simulink model "tb_elec_plant"  (R2026b)
values from neighbouring files (symbols this model uses):
  P = evalin('base', 'P')    [elec_harness.m]    (also in mcu_can1_roundtrip.m; mcu_can2_roundtrip.m; mcu_cl_input.m; mcu_ctrl_harness.m)
  Ts = prm(1)    [mcu_cl_track_dyn.m]    (also in mcu_ctrl_harness.m = evalin('base', tsExpr))
undefined symbols (not defined in the file or in its folder): EStop_Ch1_OK, EStop_Ch2_OK, G_solar, K1_Closed, K2_Closed, Key_On, Rail_12V_OK, Rail_24V_OK, Rail_3V3_OK, Rail_5V_OK, Safety_HV_OK, Safety_OK, T_amb, V_12V_V, V_24V_V, V_3V3_V, V_5V_V, V_bus_V, V_pack_V
settings Model: Creator=aomar  LastModifiedBy=aomar

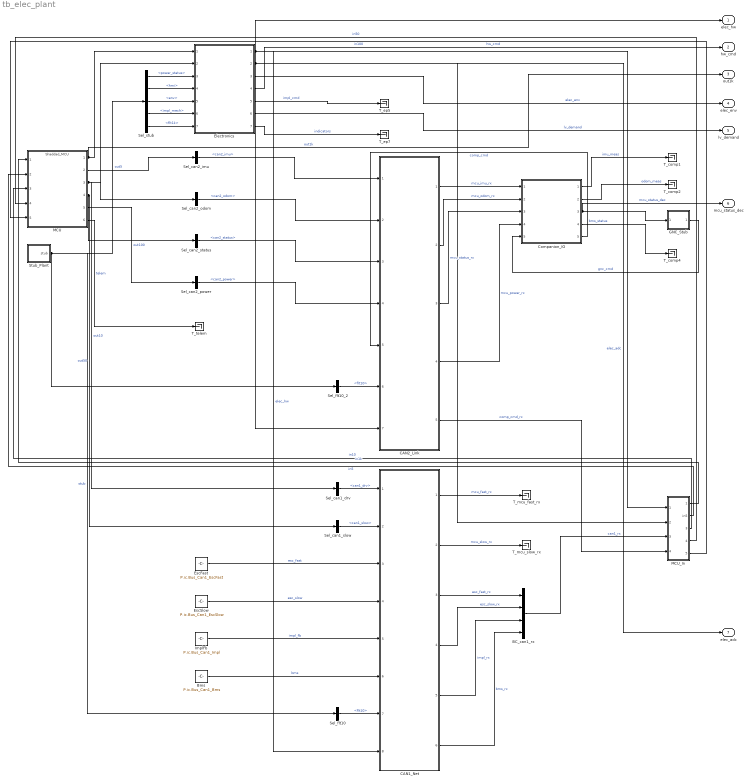
== system tb_elec_plant ==
  BC_can1_rx : BusCreator  Inputs=4
  Bms : Constant  Value=P.ic.Bus_Can1_Bms  OutDataTypeStr=Bus: Bus_Can1_Bms  SampleTime=Ts.hk
  CAN1_Net : Subsystem  ReferencedSubsystem=CAN1_Net_Sim
  CAN2_Link : Subsystem  ReferencedSubsystem=Link_MCU_GNC
  Companion_IO : Subsystem  ReferencedSubsystem=companion_io
  Electronics : Subsystem  ReferencedSubsystem=Electronics_Plant
  EscFast : Constant  Value=P.ic.Bus_Can1_EscFast  OutDataTypeStr=Bus: Bus_Can1_EscFast  SampleTime=Ts.ctrl
  EscSlow : Constant  Value=P.ic.Bus_Can1_EscSlow  OutDataTypeStr=Bus: Bus_Can1_EscSlow  SampleTime=Ts.comm
  GNC_Stub : Subsystem
  ImplFb : Constant  Value=P.ic.Bus_Can1_Impl  OutDataTypeStr=Bus: Bus_Can1_Impl  SampleTime=Ts.comm
  MCU : ModelReference  ModelNameDialog=Shaddad_MCU  SimulationMode=Normal  ModelReferenceVersion=1.1
  MCU_In : Subsystem
  Sel_can1_drv : BusSelector  OutputSignals=can1_drv
  Sel_can1_slow : BusSelector  OutputSignals=can1_slow
  Sel_can2_imu : BusSelector  OutputSignals=can2_imu
  Sel_can2_odom : BusSelector  OutputSignals=can2_odom
  Sel_can2_power : BusSelector  OutputSignals=can2_power
  Sel_can2_status : BusSelector  OutputSignals=can2_status
  Sel_flt10 : BusSelector  OutputSignals=flt10
  Sel_flt10_2 : BusSelector  OutputSignals=flt10
  Sel_stub : BusSelector  OutputSignals=power_status,hmi,env,impl_mech,flt1k
  Stub_Plant : Subsystem
  T_comp1 : Terminator
  T_comp2 : Terminator
  T_comp4 : Terminator
  T_ep5 : Terminator
  T_ep7 : Terminator
  T_mcu_fast_rx : Terminator
  T_mcu_slow_rx : Terminator
  T_telem : Terminator
  elec_hw : Outport  OutDataTypeStr=Bus: Bus_ElecHwIn
  hw_cmd : Outport  Port=2  OutDataTypeStr=Bus: Bus_PowerHwCmd
  out1k : Outport  Port=3  OutDataTypeStr=Bus: Bus_McuOut1k
  elec_env : Outport  Port=4  OutDataTypeStr=Bus: Bus_ElecEnv
  lv_demand : Outport  Port=5  OutDataTypeStr=Bus: Bus_LV_LoadDemand
  mcu_status_dec : Outport  Port=6  OutDataTypeStr=Bus: Bus_McuStatus
  elec_adc : Outport  Port=7  OutDataTypeStr=Bus: Bus_ElecAdc
  wires:
  Stub_Plant/1(stub) -> Sel_flt10/1, Sel_stub/1, Sel_flt10_2/1  "stub"
  MCU/1 -> Electronics/1, out1k/1  "out1k"
  MCU/2 -> Sel_can2_imu/1  "out5"
  MCU/5 -> Sel_can2_power/1  "out100"
  MCU/6 -> T_telem/1  "telem"
  Sel_stub/1 -> Electronics/3  "<power_status>"
  Sel_stub/2 -> Electronics/4  "<hmi>"
  Sel_stub/3 -> Electronics/5  "<env>"
  Sel_stub/4 -> Electronics/6  "<impl_mech>"
  Sel_stub/5 -> Electronics/7  "<flt1k>"
  Sel_can2_imu/1 -> CAN2_Link/1  "<can2_imu>"
  Sel_can2_odom/1 -> CAN2_Link/2  "<can2_odom>"
  Sel_can2_status/1 -> CAN2_Link/3  "<can2_status>"
  Sel_can2_power/1 -> CAN2_Link/4  "<can2_power>"
  EscFast/1 -> CAN1_Net/3  "esc_fast"
  EscSlow/1 -> CAN1_Net/4  "esc_slow"
  ImplFb/1 -> CAN1_Net/5  "impl_fb"
  Bms/1 -> CAN1_Net/6  "bms"
  Electronics/1 -> CAN1_Net/8, MCU_In/1(elec_hw), CAN2_Link/7, elec_hw/1  "elec_hw"
  Electronics/2 -> elec_adc/1, MCU_In/2(elec_adc)  "elec_adc"
  Electronics/3 -> elec_env/1  "elec_env"
  Electronics/4 -> hw_cmd/1  "hw_cmd"
  Electronics/5 -> T_ep5/1  "impl_cmd"
  Electronics/6 -> lv_demand/1  "lv_demand"
  Electronics/7 -> T_ep7/1  "indicators"
  Sel_flt10_2/1 -> CAN2_Link/6  "<flt10>"
  Sel_can1_drv/1 -> CAN1_Net/1  "<can1_drv>"
  Sel_can1_slow/1 -> CAN1_Net/2  "<can1_slow>"
  Sel_flt10/1 -> CAN1_Net/7  "<flt10>"
  CAN2_Link/1 -> Companion_IO/1  "mcu_imu_rx"
  CAN2_Link/2 -> Companion_IO/2  "mcu_odom_rx"
  CAN2_Link/3 -> Companion_IO/3  "mcu_status_rx"
  CAN2_Link/4 -> Companion_IO/4  "mcu_power_rx"
  CAN2_Link/5 -> MCU_In/4(comp)  "comp_cmd_rx"
  CAN1_Net/1 -> T_mcu_fast_rx/1  "mcu_fast_rx"
  CAN1_Net/2 -> T_mcu_slow_rx/1  "mcu_slow_rx"
  CAN1_Net/3 -> BC_can1_rx/1  "esc_fast_rx"
  CAN1_Net/4 -> BC_can1_rx/2  "esc_slow_rx"
  CAN1_Net/5 -> BC_can1_rx/3  "impl_rx"
  CAN1_Net/6 -> BC_can1_rx/4  "bms_rx"
  BC_can1_rx/1 -> MCU_In/3(can1)  "can1_rx"
  Companion_IO/1 -> T_comp1/1  "imu_meas"
  Companion_IO/2 -> T_comp2/1  "odom_meas"
  Companion_IO/3 -> GNC_Stub/1(mcu_status), mcu_status_dec/1  "mcu_status_dec"
  Companion_IO/4 -> T_comp4/1  "bms_status"
  Companion_IO/5 -> CAN2_Link/5  "comp_cmd"
  GNC_Stub/1(gnc_cmd) -> Companion_IO/5  "gnc_cmd"
  MCU_In/1(in1k) -> MCU/1  "in1k"
  MCU_In/2(in5) -> MCU/2  "in5"
  MCU_In/3(in10) -> MCU/3  "in10"
  MCU_In/4(in50) -> MCU/4  "in50"
  MCU_In/5(in100) -> MCU/5  "in100"
  MCU/3 -> Sel_can1_drv/1, Electronics/2, Sel_can2_odom/1  "out10"
  MCU/4 -> Sel_can1_slow/1, Sel_can2_status/1  "out50"

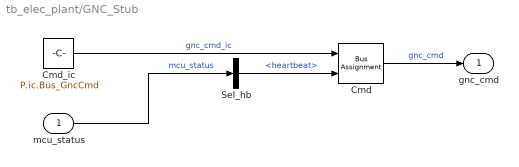
== system tb_elec_plant/GNC_Stub ==
  mcu_status : Inport
  Cmd : BusAssignment  AssignedSignals=seq
  Cmd_ic : Constant  Value=P.ic.Bus_GncCmd  OutDataTypeStr=Bus: Bus_GncCmd  SampleTime=Ts.comm
  Sel_hb : BusSelector  OutputSignals=heartbeat
  gnc_cmd : Outport
  wires:
  Cmd_ic/1 -> Cmd/1  "gnc_cmd_ic"
  mcu_status/1 -> Sel_hb/1  "mcu_status"
  Sel_hb/1 -> Cmd/2  "<heartbeat>"
  Cmd/1 -> gnc_cmd/1  "gnc_cmd"

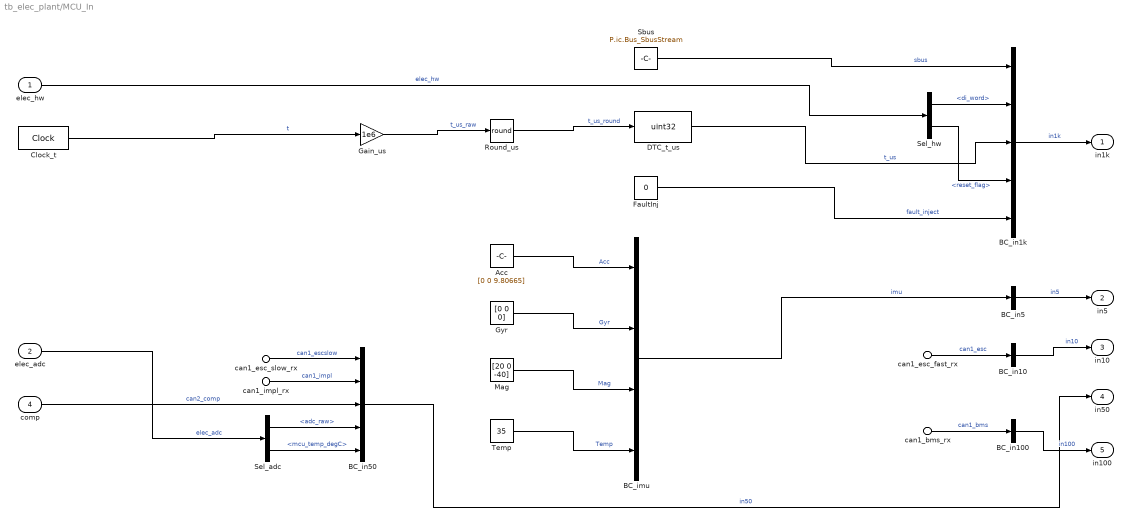
== system tb_elec_plant/MCU_In ==
  elec_hw : Inport
  elec_adc : Inport  Port=2
  can1_esc_fast_rx : Inport  Port=3  PortName=can1  Element=esc_fast_rx
  can1_esc_slow_rx : Inport  Port=3  PortName=can1  Element=esc_slow_rx
  can1_impl_rx : Inport  Port=3  PortName=can1  Element=impl_rx
  can1_bms_rx : Inport  Port=3  PortName=can1  Element=bms_rx
  comp : Inport  Port=4
  Acc : Constant  Value=[0 0 9.80665]  OutDataTypeStr=single  SampleTime=Ts.imu
  BC_imu : BusCreator  Inputs=4  OutDataTypeStr=Bus: Bus_ImuRaw  NonVirtualBus=on
      settings: InheritFromInputs=off
  BC_in10 : BusCreator  Inputs=1  OutDataTypeStr=Bus: Bus_McuIn10  NonVirtualBus=on
      settings: InheritFromInputs=off
  BC_in100 : BusCreator  Inputs=1  OutDataTypeStr=Bus: Bus_McuIn100  NonVirtualBus=on
      settings: InheritFromInputs=off
  BC_in1k : BusCreator  Inputs=5  OutDataTypeStr=Bus: Bus_McuIn1k  NonVirtualBus=on
      settings: InheritFromInputs=off
  BC_in5 : BusCreator  Inputs=1  OutDataTypeStr=Bus: Bus_McuIn5  NonVirtualBus=on
      settings: InheritFromInputs=off
  BC_in50 : BusCreator  Inputs=5  OutDataTypeStr=Bus: Bus_McuIn50  NonVirtualBus=on
      settings: InheritFromInputs=off
  Clock_t : DigitalClock  SampleTime=Ts.base
  DTC_t_us : DataTypeConversion  OutDataTypeStr=uint32  SaturateOnIntegerOverflow=off  RndMeth=Floor
  FaultInj : Constant  Value=0  OutDataTypeStr=uint32  SampleTime=Ts.base
  Gain_us : Gain  Gain=1e6
  Gyr : Constant  Value=[0 0 0]  OutDataTypeStr=single  SampleTime=Ts.imu
  Mag : Constant  Value=[20 0 -40]  OutDataTypeStr=single  SampleTime=Ts.imu
  Round_us : Rounding  Operator=round
  Sbus : Constant  Value=P.ic.Bus_SbusStream  OutDataTypeStr=Bus: Bus_SbusStream  SampleTime=Ts.base
  Sel_adc : BusSelector  OutputSignals=adc_raw,mcu_temp_degC
  Sel_hw : BusSelector  OutputSignals=di_word,reset_flag
  Temp : Constant  Value=35  OutDataTypeStr=single  SampleTime=Ts.imu
  in1k : Outport
  in5 : Outport  Port=2
  in10 : Outport  Port=3
  in50 : Outport  Port=4
  in100 : Outport  Port=5
  wires:
  elec_hw/1 -> Sel_hw/1  "elec_hw"
  elec_adc/1 -> Sel_adc/1  "elec_adc"
  comp/1 -> BC_in50/3  "can2_comp"
  Clock_t/1 -> Gain_us/1  "t"
  can1_esc_slow_rx/1 -> BC_in50/1  "can1_escslow"
  can1_impl_rx/1 -> BC_in50/2  "can1_impl"
  Sel_adc/1 -> BC_in50/4  "<adc_raw>"
  Sel_adc/2 -> BC_in50/5  "<mcu_temp_degC>"
  BC_in50/1 -> in50/1  "in50"
  Gain_us/1 -> Round_us/1  "t_us_raw"
  Round_us/1 -> DTC_t_us/1  "t_us_round"
  Acc/1 -> BC_imu/1  "Acc"
  Gyr/1 -> BC_imu/2  "Gyr"
  Mag/1 -> BC_imu/3  "Mag"
  Temp/1 -> BC_imu/4  "Temp"
  BC_imu/1 -> BC_in5/1  "imu"
  Sbus/1 -> BC_in1k/1  "sbus"
  FaultInj/1 -> BC_in1k/5  "fault_inject"
  DTC_t_us/1 -> BC_in1k/3  "t_us"
  Sel_hw/1 -> BC_in1k/2  "<di_word>"
  Sel_hw/2 -> BC_in1k/4  "<reset_flag>"
  can1_esc_fast_rx/1 -> BC_in10/1  "can1_esc"
  can1_bms_rx/1 -> BC_in100/1  "can1_bms"
  BC_in1k/1 -> in1k/1  "in1k"
  BC_in5/1 -> in5/1  "in5"
  BC_in10/1 -> in10/1  "in10"
  BC_in100/1 -> in100/1  "in100"

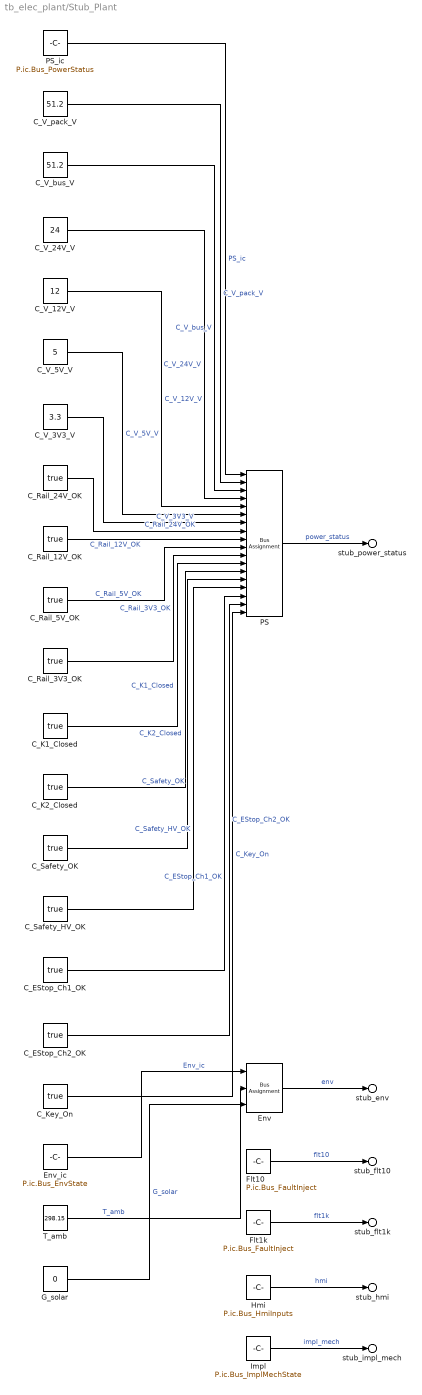
== system tb_elec_plant/Stub_Plant ==
  C_EStop_Ch1_OK : Constant  Value=true  OutDataTypeStr=boolean  SampleTime=Ts.base
  C_EStop_Ch2_OK : Constant  Value=true  OutDataTypeStr=boolean  SampleTime=Ts.base
  C_K1_Closed : Constant  Value=true  OutDataTypeStr=boolean  SampleTime=Ts.base
  C_K2_Closed : Constant  Value=true  OutDataTypeStr=boolean  SampleTime=Ts.base
  C_Key_On : Constant  Value=true  OutDataTypeStr=boolean  SampleTime=Ts.base
  C_Rail_12V_OK : Constant  Value=true  OutDataTypeStr=boolean  SampleTime=Ts.base
  C_Rail_24V_OK : Constant  Value=true  OutDataTypeStr=boolean  SampleTime=Ts.base
  C_Rail_3V3_OK : Constant  Value=true  OutDataTypeStr=boolean  SampleTime=Ts.base
  C_Rail_5V_OK : Constant  Value=true  OutDataTypeStr=boolean  SampleTime=Ts.base
  C_Safety_HV_OK : Constant  Value=true  OutDataTypeStr=boolean  SampleTime=Ts.base
  C_Safety_OK : Constant  Value=true  OutDataTypeStr=boolean  SampleTime=Ts.base
  C_V_12V_V : Constant  Value=12  OutDataTypeStr=double  SampleTime=Ts.base
  C_V_24V_V : Constant  Value=24  OutDataTypeStr=double  SampleTime=Ts.base
  C_V_3V3_V : Constant  Value=3.3  OutDataTypeStr=double  SampleTime=Ts.base
  C_V_5V_V : Constant  Value=5  OutDataTypeStr=double  SampleTime=Ts.base
  C_V_bus_V : Constant  Value=51.2  OutDataTypeStr=double  SampleTime=Ts.base
  C_V_pack_V : Constant  Value=51.2  OutDataTypeStr=double  SampleTime=Ts.base
  Env : BusAssignment  AssignedSignals=T_amb,G_solar
  Env_ic : Constant  Value=P.ic.Bus_EnvState  OutDataTypeStr=Bus: Bus_EnvState  SampleTime=Ts.hk
  Flt10 : Constant  Value=P.ic.Bus_FaultInject  OutDataTypeStr=Bus: Bus_FaultInject  SampleTime=Ts.ctrl
  Flt1k : Constant  Value=P.ic.Bus_FaultInject  OutDataTypeStr=Bus: Bus_FaultInject  SampleTime=Ts.base
  G_solar : Constant  Value=0  OutDataTypeStr=double  SampleTime=Ts.hk
  Hmi : Constant  Value=P.ic.Bus_HmiInputs  OutDataTypeStr=Bus: Bus_HmiInputs  SampleTime=Ts.base
  Impl : Constant  Value=P.ic.Bus_ImplMechState  OutDataTypeStr=Bus: Bus_ImplMechState  SampleTime=Ts.ctrl
  PS : BusAssignment  AssignedSignals=V_pack_V,V_bus_V,V_24V_V,V_12V_V,V_5V_V,V_3V3_V,Rail_24V_OK,Rail_12V_OK,Rail_5V_OK,Rail_3V3_OK,K1_Closed,K2_Closed,Safety_OK,Safety_HV_OK,EStop_Ch1_OK,EStop_Ch2_OK,Key_On
  PS_ic : Constant  Value=P.ic.Bus_PowerStatus  OutDataTypeStr=Bus: Bus_PowerStatus  SampleTime=Ts.base
  T_amb : Constant  Value=298.15  OutDataTypeStr=double  SampleTime=Ts.hk
  stub_power_status : Outport  PortName=stub  Element=power_status
  stub_hmi : Outport  PortName=stub  Element=hmi
  stub_env : Outport  PortName=stub  Element=env
  stub_impl_mech : Outport  PortName=stub  Element=impl_mech
  stub_flt1k : Outport  PortName=stub  Element=flt1k
  stub_flt10 : Outport  PortName=stub  Element=flt10
  wires:
  PS_ic/1 -> PS/1  "PS_ic"
  C_V_pack_V/1 -> PS/2  "C_V_pack_V"
  C_V_bus_V/1 -> PS/3  "C_V_bus_V"
  C_V_24V_V/1 -> PS/4  "C_V_24V_V"
  C_V_12V_V/1 -> PS/5  "C_V_12V_V"
  C_V_5V_V/1 -> PS/6  "C_V_5V_V"
  C_V_3V3_V/1 -> PS/7  "C_V_3V3_V"
  C_Rail_24V_OK/1 -> PS/8  "C_Rail_24V_OK"
  C_Rail_12V_OK/1 -> PS/9  "C_Rail_12V_OK"
  C_Rail_5V_OK/1 -> PS/10  "C_Rail_5V_OK"
  C_Rail_3V3_OK/1 -> PS/11  "C_Rail_3V3_OK"
  C_K1_Closed/1 -> PS/12  "C_K1_Closed"
  C_K2_Closed/1 -> PS/13  "C_K2_Closed"
  C_Safety_OK/1 -> PS/14  "C_Safety_OK"
  C_Safety_HV_OK/1 -> PS/15  "C_Safety_HV_OK"
  C_EStop_Ch1_OK/1 -> PS/16  "C_EStop_Ch1_OK"
  C_EStop_Ch2_OK/1 -> PS/17  "C_EStop_Ch2_OK"
  C_Key_On/1 -> PS/18  "C_Key_On"
  Env_ic/1 -> Env/1  "Env_ic"
  T_amb/1 -> Env/2  "T_amb"
  G_solar/1 -> Env/3  "G_solar"
  Flt10/1 -> stub_flt10/1  "flt10"
  Flt1k/1 -> stub_flt1k/1  "flt1k"
  Hmi/1 -> stub_hmi/1  "hmi"
  Impl/1 -> stub_impl_mech/1  "impl_mech"
  PS/1 -> stub_power_status/1  "power_status"
  Env/1 -> stub_env/1  "env"
